simulink model "rfdc"  (R2019a)
settings: Solver=VariableStepAuto  StartTime=0.0  StopTime=10.0  RelTol=1e-3
libraries: xbsIndex_r4 x6
(part 2 of 2)

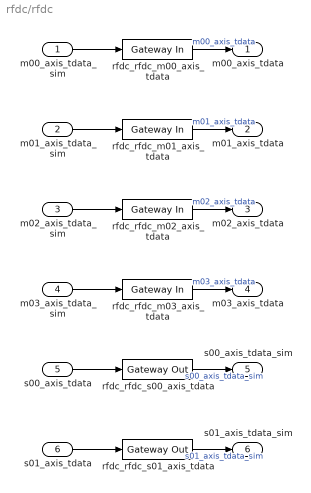
== system rfdc/rfdc ==
  m00_axis_tdata_sim : Inport
  m01_axis_tdata_sim : Inport  Port=2
  m02_axis_tdata_sim : Inport  Port=3
  m03_axis_tdata_sim : Inport  Port=4
  s00_axis_tdata : Inport  Port=5
  s01_axis_tdata : Inport  Port=6
  rfdc_rfdc_m00_axis_tdata : xbsIndex_r4/Gateway In  gui_display_data_type=Fixed-point  arith_type="Signed  (2's comp)"  n_bits=64  bin_pt=0  preci_type=Single  exp_width=8  frac_width=24  rows=1  columns=1  quantization="Round  (unbiased: +/- Inf)"  overflow=Saturate  period=1  UseAsADC=off  ADCChannel='1'  interface=None  automatic_assignment=on  address_offset=hex2dec('00')  intf_name=''  intf_description=''  default_value=0  timing_constraint=None  locs_specified=off  LOCs={}  io_standard={}  inherit_from_input=off  hdl_port=on  dbl_ovrd=off  block_type=gatewayin
  rfdc_rfdc_m01_axis_tdata : xbsIndex_r4/Gateway In  gui_display_data_type=Fixed-point  arith_type="Signed  (2's comp)"  n_bits=64  bin_pt=0  preci_type=Single  exp_width=8  frac_width=24  rows=1  columns=1  quantization="Round  (unbiased: +/- Inf)"  overflow=Saturate  period=1  UseAsADC=off  ADCChannel='1'  interface=None  automatic_assignment=on  address_offset=hex2dec('00')  intf_name=''  intf_description=''  default_value=0  timing_constraint=None  locs_specified=off  LOCs={}  io_standard={}  inherit_from_input=off  hdl_port=on  dbl_ovrd=off  block_type=gatewayin
  rfdc_rfdc_m02_axis_tdata : xbsIndex_r4/Gateway In  gui_display_data_type=Fixed-point  arith_type="Signed  (2's comp)"  n_bits=64  bin_pt=0  preci_type=Single  exp_width=8  frac_width=24  rows=1  columns=1  quantization="Round  (unbiased: +/- Inf)"  overflow=Saturate  period=1  UseAsADC=off  ADCChannel='1'  interface=None  automatic_assignment=on  address_offset=hex2dec('00')  intf_name=''  intf_description=''  default_value=0  timing_constraint=None  locs_specified=off  LOCs={}  io_standard={}  inherit_from_input=off  hdl_port=on  dbl_ovrd=off  block_type=gatewayin
  rfdc_rfdc_m03_axis_tdata : xbsIndex_r4/Gateway In  gui_display_data_type=Fixed-point  arith_type="Signed  (2's comp)"  n_bits=64  bin_pt=0  preci_type=Single  exp_width=8  frac_width=24  rows=1  columns=1  quantization="Round  (unbiased: +/- Inf)"  overflow=Saturate  period=1  UseAsADC=off  ADCChannel='1'  interface=None  automatic_assignment=on  address_offset=hex2dec('00')  intf_name=''  intf_description=''  default_value=0  timing_constraint=None  locs_specified=off  LOCs={}  io_standard={}  inherit_from_input=off  hdl_port=on  dbl_ovrd=off  block_type=gatewayin
  rfdc_rfdc_s00_axis_tdata : xbsIndex_r4/Gateway Out  inherit_from_input=off  hdl_port=on  rows=1  columns=1  UseAsDAC=off  DACChannel='1'  interface=None  automatic_assignment=on  address_offset=hex2dec('00')  intf_name=''  intf_description=''  timing_constraint=None  locs_specified=off  LOCs={}  io_standard={}  block_type=gatewayout
  rfdc_rfdc_s01_axis_tdata : xbsIndex_r4/Gateway Out  inherit_from_input=off  hdl_port=on  rows=1  columns=1  UseAsDAC=off  DACChannel='1'  interface=None  automatic_assignment=on  address_offset=hex2dec('00')  intf_name=''  intf_description=''  timing_constraint=None  locs_specified=off  LOCs={}  io_standard={}  block_type=gatewayout
  m00_axis_tdata : Outport
  m01_axis_tdata : Outport  Port=2
  m02_axis_tdata : Outport  Port=3
  m03_axis_tdata : Outport  Port=4
  s00_axis_tdata_sim : Outport  Port=5
  s01_axis_tdata_sim : Outport  Port=6
  wires:
  m00_axis_tdata_sim/1 -> rfdc_rfdc_m00_axis_tdata/1
  rfdc_rfdc_m00_axis_tdata/1 -> m00_axis_tdata/1  "m00_axis_tdata"
  m01_axis_tdata_sim/1 -> rfdc_rfdc_m01_axis_tdata/1
  rfdc_rfdc_m01_axis_tdata/1 -> m01_axis_tdata/1  "m01_axis_tdata"
  m02_axis_tdata_sim/1 -> rfdc_rfdc_m02_axis_tdata/1
  rfdc_rfdc_m02_axis_tdata/1 -> m02_axis_tdata/1  "m02_axis_tdata"
  m03_axis_tdata_sim/1 -> rfdc_rfdc_m03_axis_tdata/1
  rfdc_rfdc_m03_axis_tdata/1 -> m03_axis_tdata/1  "m03_axis_tdata"
  s00_axis_tdata/1 -> rfdc_rfdc_s00_axis_tdata/1
  rfdc_rfdc_s00_axis_tdata/1 -> s00_axis_tdata_sim/1  "s00_axis_tdata_sim"
  s01_axis_tdata/1 -> rfdc_rfdc_s01_axis_tdata/1
  rfdc_rfdc_s01_axis_tdata/1 -> s01_axis_tdata_sim/1  "s01_axis_tdata_sim"
